simulink model "projectsubaslxcorr"  (R2025a)
settings: Solver=FixedStepAuto  StartTime=0.0  StopTime=0.5  FixedStep=2e-6  RelTol=1e-3
undefined symbols (not defined in the file): dspblkCoreblockFVToolHelper, gcbh
libraries: nesl_utility x21, fl_lib x18, ee_lib x5, simulink x5
settings Model: Creator=Loganathan Mukundhan  LastModifiedBy=msssr

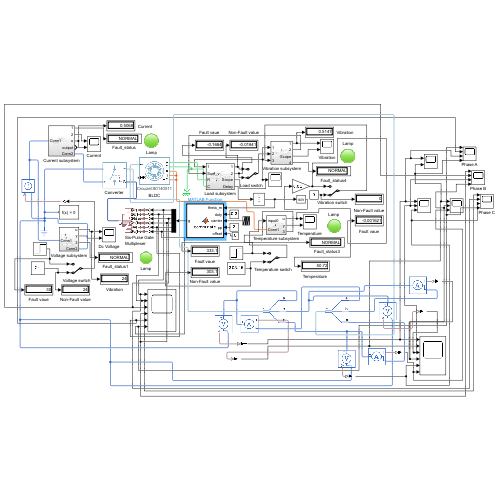
[thumbnail: Simulink's stored preview of the top-level diagram]
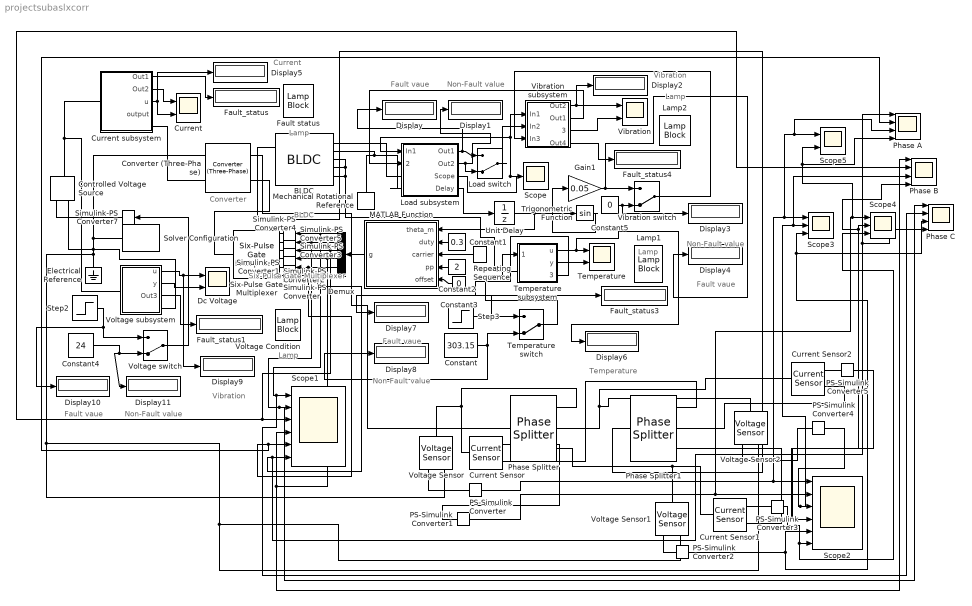
== system projectsubaslxcorr ==
  note: Vibration
  note: Current
  note: Vibration
  note: Fault vaue
  note: Non-Fault value
  note: Temperature
  note: Converter
  note: Six-Pulse Gate
      | Multiplexer
  note: BLDC
  note: Lamp
  note: Lamp
  note: Lamp
  note: Lamp
  note: Non-Fault value
  note: Fault vaue
  note: Non-Fault value
  note: Fault vaue
  note: Non-Fault value
  note: Fault vaue
  BLDC : ee_lib/Electromechanical/Permanent Magnet/BLDC  PartSpecification="{\"CollectionId\":\"SimscapeElectrical\",\"CollectionVersion\":\"1.0.0\",\"DatasetId\":\"Crouzet|80140511|simscape.electrical.bldc\",\"DisplayName\":\"Crouzet:80140511\"}"  port_option=ee.enum.threePhasePort.composite  rotor_param=ee.enum.pmsm.backemf.trapezoidflux  pm_flux_linkage=0.0384885225157163 % Datasheet derived Wb  theta_constant=60 % Assumed angle deg  emf_max=9.6 % Parameter not set V  w_meas=600 % Parameter not set rpm  DphiDtheta_tab=[0, -.1528, -.1528, .1528, .1528, 0] % Parameter not set Wb/rad  back_emf_tab=[0, -9.6, -9.6, 9.6, 9.6, 0] % Parameter not set V  rotor_angle_tab=[0, 7.5, 22.5, 37.5, 52.5, 60] % Parameter not set deg  nPolePairs=2 % Datasheet derived  axes_param=ee.enum.rotorangle.qaxis  winding_type=ee.enum.statorconnection.delta  stator_param=ee.enum.statorparam.LdLqL0  machine_param=ee.enum.dqparameterization.constant  Ld=3.15 % Datasheet derived mH  Lq=3.15 % Datasheet derived mH  idVec=[-200, 0, 200] % Parameter not set A  iqVec=[-200, 0, 200] % Parameter not set A  LdMatrix=0.00022 * ones(3, 3) % Parameter not set H  LqMatrix=0.00022 * ones(3, 3) % Parameter not set H  L0=3.15 % Assumed inductance value mH  Ls=Ls % Parameter not set H  Lm=0 % Parameter not set H  Ms=Ms % Parameter not set H  Rs=1.545 % Datasheet derived Ohm  zero_sequence=ee.enum.park.zerosequence.exclude  loss_param=ee.enum.ironloss.none  losses_oc=[0, 0, 0] % Parameter not set W  losses_sc=[0, 0, 0] % Parameter not set W  f_losses=60 % Parameter not set Hz  Isc_losses=95 % Parameter not set A  J=5e-06 % Datasheet derived kg*m^2  lam=0 % Parameter not set N*m/(rad/s)  i_d_specify=off  i_d_priority=None  i_d=0 A  i_d_nominal_specify=off  i_d_nominal_value=1  i_d_nominal_unit=A  i_q_specify=off  i_q_priority=None  i_q=0 A  i_q_nominal_specify=off  i_q_nominal_value=1  i_q_nominal_unit=A  torque_specify=off  torque_priority=None  torque=0 N*m  torque_nominal_specify=off  torque_nominal_value=1  torque_nominal_unit=N*m  angular_velocity_specify=off  angular_velocity_priority=High  angular_velocity=0 rpm  angular_velocity_nominal_specify=off  angular_velocity_nominal_value=1  angular_velocity_nominal_unit=rpm  angular_position_specify=off  angular_position_priority=High  angular_position=0 deg  angular_position_nominal_specify=off  angular_position_nominal_value=1  angular_position_nominal_unit=deg  alpha=0.00393 % Parameter not set 1/K  alpha_flux=-0.001 % Parameter not set 1/K  Tmeas=298.15 % Parameter not set K  stator_thermal_mass=0.02 J/K  rotor_thermal_mass=0.05 J/K  Rm_percent_rotor=90  Rd_percent_rotor=30  temperatureA_specify=off  temperatureA_priority=High  temperatureA=25 degC  temperatureA_nominal_specify=off  temperatureA_nominal_value=1  temperatureA_nominal_unit=degC  temperatureB_specify=off  temperatureB_priority=High  temperatureB=25 degC  temperatureB_nominal_specify=off  temperatureB_nominal_value=1  temperatureB_nominal_unit=degC  temperatureC_specify=off  temperatureC_priority=High  temperatureC=25 degC  temperatureC_nominal_specify=off  temperatureC_nominal_value=1  temperatureC_nominal_unit=degC  temperatureR_specify=off  temperatureR_priority=High  temperatureR=25 degC  temperatureR_nominal_specify=off  temperatureR_nominal_value=1  temperatureR_nominal_unit=degC
      settings: AttributesFormatString=Crouzet:80140511  InternalSimscapePortConfiguration="{\"Bottom\":[],\"Left\":[{\"id\":\"N\",\"label\":\"~\",\"type\":\"foundation.electrical.three_phase\"},{\"id\":\"HR\",\"label\":\"HR\",\"type\":\"foundation.thermal.thermal\"}],\"Right\":[{\"id\":\"R\",\"label\":\"R\",\"type\":\"foundation.mechanical.rotational.rotational\"},{\"id\":\"C\",\"label\":\"C\",\"type\":\"foundation.mechanical.rotational.rotational\"},{\"id\":\"HA\",\"label\":\"HA\",\"type\":\"foundation.thermal.thermal\"},{\"id\":\"HB\",\"label\":\"HB\",\"type\":\"foundation.thermal.thermal\"},{\"id\":\"HC\",\"label\":\"HC\",\"type\":\"foundation.thermal.thermal\"}],\"Top\":[]}"
  Constant : Constant  Value=303.15
  Constant1 : Constant  Value=0.3
  Constant2 : Constant  Value=2
  Constant3 : Constant  Value=0
  Constant4 : Constant  Value=24
  Constant5 : Constant  Value=0
  Controlled Voltage Source : fl_lib/Electrical/Electrical Sources/Controlled Voltage Source
  Converter (Three-Phase) : ee_lib/Semiconductors & Converters/Converters/Converter (Three-Phase)  port_option=ee.enum.threePhasePort.composite  fidelity_option=ee.enum.converters.fidelity.detailed  device_type=ee.enum.converters.switchingdevice.mosfet  showThermalPort=false  K=0  Vth=0.5 V  Vgt=1 V  Vgt_off=-1 V  Ih=1 A  Vf=0.8 V  Ron=0.001 Ohm  Rds=0.001 Ohm  Goff=1e-6 1/Ohm  Eon_scalar=22.86e-3 J  Eoff_scalar=17.14e-3 J  Eoff_natural_commutation=10e-3 J  Voff=300 V  Iout_scalar=600 A  onCurrentMeasDelay=0 s  useCurrentFromPreviousCycle=false  useVoltageFromPreviousCycle=false  diode_param=ee.enum.converters.protectiondiode.nodynamics  diode_Vf=0.8 V  diode_Ron=0.001 Ohm  diode_Goff=1e-5 1/Ohm  diode_C=50 nF  diode_iRM=-235 A  diode_iF=300 A  diode_idot=-50 A/us  diode_trr_param=ee.enum.converters.diodetrr.trr_factor  diode_trr_factor=3  diode_trr=15 us  diode_Qrr=1500 s*uA  diode_rec_loss_model=ee.enum.diode.reverseRecoveryModel.fixed  diode_ErecVal=0 J  diode_scaleWithIandV=false  diode_ErecMat=zeros(2, 3) J  diode_TjrecVec=[298.15, 398.15] K  diode_IfrecVec=[.1, 1, 10] A  diode_IrecVal=10 A  diode_VrecVal=10 V  diode_tFilter=1 / 1000 / 100 s  thermal_network_parameterization=ee.enum.thermalNetworkTopology.external  Rth=[.08, .5] K/W  Rth_Cauer=[.08, .1, .5] K/W  Rth_Foster=[.08, .14, .22, .16] K/W  thermal_mass_parameterization=ee.enum.thermalNetwork.timeconstant  thermal_mass=[.01, .5] J/K  thermal_mass_Cauer=[.01, .1, .5] J/K  thermal_mass_Foster=[.001, .005, .05, .5] J/K  thermal_time_constant=[.001, .2] s  thermal_time_constant_Cauer=[.001, .1, .2] s  thermal_time_constant_Foster=[7e-05, .0007, .01, .08] s  thermal_mass_initial_temperatures=[25, 25] degC  thermal_mass_initial_temperatures_Cauer=[25, 25, 25] degC  junction_thermal_mass=0.01 J/K  Tvec_initial_Foster=[25, 25, 25, 25] degC  snubber_type=ee.enum.converters.snubber.exclude  Cs=1e-7 F  Rs=0.1 Ohm  Vce_loss=[0, 150, 300] V
  Current : Scope  NumInputPorts=2
      settings: ActiveDisplayYMinimum=-0.12499999999999997  ActiveDisplayYMaximum=1.125  DataLoggingVariableName=ScopeData3
  Current Sensor : fl_lib/Electrical/Electrical Sensors/Current Sensor
  Current Sensor1 : fl_lib/Electrical/Electrical Sensors/Current Sensor
  Current Sensor2 : fl_lib/Electrical/Electrical Sensors/Current Sensor
  Current subsystem : Subsystem
  Dc Voltage : Scope  NumInputPorts=2
      settings: ActiveDisplayYMinimum=-1  ActiveDisplayYMaximum=1  DataLoggingVariableName=ScopeData4
  Demux : Demux  Outputs=6
  Display{,1..11} (12 alike) : Display
  Electrical Reference : fl_lib/Electrical/Electrical Elements/Electrical Reference
  Fault status : LampBlock  LabelPosition=Hide  DefaultColor=[192.0, 192.0, 192.0]
  Fault_status{,1,3..4} (4 alike) : Display
  Gain1 : Gain  Gain=0.05
  Lamp1 : LampBlock  LabelPosition=Hide  DefaultColor=[192.0, 192.0, 192.0]
  Lamp2 : LampBlock  LabelPosition=Hide  DefaultColor=[192.0, 192.0, 192.0]
  Load subsystem : Subsystem
  Load switch : ManualSwitch  CurrentSetting=0
  MATLAB Function : MATLAB Function  TreatAsAtomicUnit=on
  Mechanical Rotational Reference : fl_lib/Mechanical/Rotational Elements/Mechanical Rotational Reference
  PS-Simulink Converter{,1..5} (6 alike) : nesl_utility/PS-Simulink Converter  PhysicalDomain=network_engine_domain  SubClassName=ps_output  LeftPortType=input  RightPortType=output  PseudoPeriodic=off  Frequencies=[]  VectorFormat=inherit  Unit=inherit  AffineConversion=off
  Phase A : Scope  NumInputPorts=4
      settings: ActiveDisplayYMinimum=-0.012079831932773066  ActiveDisplayYMaximum=1.0252100840336134  DataLoggingVariableName=ScopeData10
  Phase B : Scope  NumInputPorts=4
      settings: ActiveDisplayYMinimum=-0.12499999999999997  ActiveDisplayYMaximum=1.125  DataLoggingVariableName=ScopeData11
  Phase C : Scope  NumInputPorts=4
      settings: ActiveDisplayYMinimum=-0.031775210084033612  ActiveDisplayYMaximum=1.0317752100840336  DataLoggingVariableName=ScopeData12
  Phase Splitter : ee_lib/Connectors & References/Phase Splitter
  Phase Splitter1 : ee_lib/Connectors & References/Phase Splitter
  Repeating Sequence : simulink/Sources/Repeating Sequence  rep_seq_t=[0 1e-4]  rep_seq_y=[0 1]
  Scope : Scope
      settings: ActiveDisplayYMinimum=-12.045945676542038  ActiveDisplayYMaximum=108.41351108887838
  Scope1 : Scope  NumInputPorts=6
      settings: ActiveDisplayYMinimum=-0.12499999999999997  ActiveDisplayYMaximum=1.125
  Scope2 : Scope  NumInputPorts=6
      settings: ActiveDisplayYMinimum=-1.7770072942224644  ActiveDisplayYMaximum=27.088124454668268  DataLoggingVariableName=ScopeData2
  Scope3 : Scope  NumInputPorts=3
      settings: ActiveDisplayYMinimum=-2.8282937021531112  ActiveDisplayYMaximum=26.5262867042067  DataLoggingVariableName=ScopeData5
  Scope4 : Scope  NumInputPorts=3
      settings: DataLoggingVariableName=ScopeData7
  Scope5 : Scope  NumInputPorts=2
      settings: ActiveDisplayYMinimum=-1.0622016680044801  ActiveDisplayYMaximum=26.229780400571709  DataLoggingVariableName=ScopeData9
  Simulink-PS Converter{,1..5,7} (7 alike) : nesl_utility/Simulink-PS Converter  PhysicalDomain=network_engine_domain  SubClassName=ps_input  LeftPortType=input  RightPortType=output  PseudoPeriodic=off  Frequencies=[]  NoiseDistribution=none  NoiseParameters=[]  Unit=1  AffineConversion=off  FilteringAndDerivatives=provide  SimscapeFilterOrder=1  InputFilterTimeConstant=0.001  UdotUserProvided=0
  Six-Pulse Gate Multiplexer : ee_lib/Semiconductors & Converters/Converters/Six-Pulse Gate Multiplexer  port_option=ee.enum.controlport.ps
  Solver Configuration : nesl_utility/Solver Configuration  PhysicalDomain=network_engine_domain  SubClassName=solver  LeftPortType=input  RightPortType=generic  Tones=[]  Harmonics=[]  SimulateNoise=off  Profile=off  UseLocalSampling=off  EnableSwitchedLinearOptims=on  FrequencyDomain=off  UseCCode=off  RelTol=0.001  AbsTol=0.001  MinStep=1e-09  ToWorkspace=off  RevertToSquareIcSolve=off  NumHomotopyIterations=100  PhasorMode=off  PhasorModeNumHarmonics=1  ConsistencySolver=NEWTON_XTOL_AFTER_FTOL  IndexReductionMethod=DerivativeReplacement  DoDC=off  ResidualTolerance=1e-09  ConsistencyTolSource=GLOBAL  ConsistencyAbsTol=0.001  ConsistencyRelTol=0.001  ConsistencyTolFactor=0.001  UseLocalSolver=on  LocalSolverChoice=NE_BACKWARD_EULER_ADVANCER  ResolveIndetEquations=on  FunctionEvalNumThread=1  LocalSolverSampleTime=2e-6  DoFixedCost=off  MaxNonlinIter=3  MaxModeIter=2  ComputeImpulses=off  ImpulseIterations=2  LinearAlgebra=auto  LinearAlgebraNumThread=0  EquationFormulation=NE_TIME_EF  DelaysMemoryBudget=1024  AutomaticFiltering=on  FilteringTimeConstant=0.001  PartitionStorageMethod=AS_NEEDED  PartitionMemoryBudget=1024  PartitionMethod=ROBUST  MultibodyUseLocalSolver=off  MultibodyLocalSolverChoice=ODE1  MultibodyLocalSolverSampleTime=0.001
  Step2 : Step  Time=0.25  Before=24  After=30  SampleTime=0
  Step3 : Step  Time=0.25  Before=303.15  After=333.15  SampleTime=0
  Temperature : Scope  NumInputPorts=2
      settings: ActiveDisplayYMinimum=13.049582437412266  ActiveDisplayYMaximum=132.55375806328965  DataLoggingVariableName=ScopeData6
  Temperature subsystem : Subsystem
  Temperature switch : ManualSwitch  CurrentSetting=0
  Trigonometric Function : Trigonometry
  Unit Delay : UnitDelay  SampleTime=2e-6  HasFrameUpgradeWarning=on
  Vibration : Scope  NumInputPorts=2
      settings: ActiveDisplayYMinimum=-2.0330445480545611  ActiveDisplayYMaximum=18.297400932491055  DataLoggingVariableName=ScopeData8
  Vibration subsystem : Subsystem
  "Vibration switch  " : ManualSwitch  CurrentSetting=0
  Voltage Condition : LampBlock  LabelPosition=Hide  DefaultColor=[192.0, 192.0, 192.0]
  Voltage Sensor : fl_lib/Electrical/Electrical Sensors/Voltage Sensor
  Voltage Sensor1 : fl_lib/Electrical/Electrical Sensors/Voltage Sensor
  Voltage Sensor2 : fl_lib/Electrical/Electrical Sensors/Voltage Sensor
  Voltage subsystem : Subsystem
  Voltage switch : ManualSwitch  CurrentSetting=0
  wires:
  Demux/1 -> Phase C/2, Scope1/1, Simulink-PS Converter5/1
  Demux/2 -> Phase C/1, Scope1/2, Simulink-PS Converter4/1
  Demux/3 -> Scope1/3, Phase B/2, Simulink-PS Converter3/1
  Demux/4 -> Scope1/4, Phase B/1, Simulink-PS Converter2/1
  Demux/5 -> Phase A/2, Scope1/5, Simulink-PS Converter1/1
  Demux/6 -> Phase C/4, Phase A/1, Scope1/6, Simulink-PS Converter/1
  MATLAB Function/1(g) -> Demux/1
  Constant3/1 -> MATLAB Function/5(offset)
  Constant1/1 -> MATLAB Function/2(duty)
  Constant2/1 -> MATLAB Function/4(pp)
  Repeating Sequence/1 -> MATLAB Function/3(carrier)
  Step2/1 -> Display10/1, Voltage switch/1
  Constant4/1 -> Voltage switch/2, Display11/1
  Step3/1 -> Display7/1, Temperature switch/1
  Constant/1 -> Temperature switch/2, Display8/1
  Constant5/1 -> Display3/1, "Vibration switch  "/2
  Unit Delay/1 -> Trigonometric Function/1, MATLAB Function/1(theta_m)
  Trigonometric Function/1 -> Gain1/1
  Gain1/1 -> Display4/1, "Vibration switch  "/1
  Current subsystem/1(Out1) -> Fault_status/1
  Current subsystem/2(Out2) -> Current/1
  Current subsystem/3(u) -> Current/2, Display5/1
  Voltage subsystem/1(u) -> Display9/1, Dc Voltage/1
  Voltage subsystem/3(Out3) -> Fault_status1/1
  Load subsystem/3(Scope) -> Vibration subsystem/1(In1), Load subsystem/1(In1), Scope/1
  Load subsystem/1(Out1) -> Display/1, Load switch/1
  Load subsystem/2(Out2) -> Display1/1, Load switch/2
  Load subsystem/4(Delay) -> Unit Delay/1
  Temperature switch/1 -> Temperature subsystem/1(input0)
  Temperature subsystem/1(u) -> Display6/1, Temperature/1
  Temperature subsystem/2(y) -> Temperature/2
  Temperature subsystem/3(Out3) -> Fault_status3/1
  Load switch/1 -> Vibration subsystem/2(In2)
  "Vibration switch  "/1 -> Vibration subsystem/3(In3)
  Vibration subsystem/2(Out1) -> Load subsystem/2(Sum_v)
  Vibration subsystem/1(Out2) -> Vibration/1, Display2/1
  Vibration subsystem/3(Scope) -> Vibration/2
  Vibration subsystem/4(Out4) -> Fault_status4/1
  Voltage switch/1 -> Simulink-PS Converter7/1
  Voltage subsystem/2(y) -> Dc Voltage/2
  PS-Simulink Converter/1 -> Phase A/3, Scope5/1, Scope3/1, Scope2/1
  PS-Simulink Converter1/1 -> Scope2/2, Phase A/4, Scope5/2, Scope4/1
  PS-Simulink Converter4/1 -> Phase B/3, Scope3/2, Scope2/3
  PS-Simulink Converter5/1 -> Scope2/4, Scope4/2, Phase B/4
  PS-Simulink Converter2/1 -> Scope2/5, Phase C/3, Scope3/3
  PS-Simulink Converter3/1 -> Scope4/3, Scope2/6
  connections:
  Solver Configuration/RConn1 -- Voltage Sensor1/RConn2 -- Voltage Sensor2/RConn2 -- Voltage Sensor/RConn2 -- Electrical Reference/LConn1 -- Controlled Voltage Source/RConn2 -- Voltage subsystem/RConn1 -- Converter (Three-Phase)/RConn2
  Six-Pulse Gate Multiplexer/RConn1 -- Converter (Three-Phase)/LConn1
  Simulink-PS Converter5/RConn1 -- Six-Pulse Gate Multiplexer/LConn6
  Simulink-PS Converter4/RConn1 -- Six-Pulse Gate Multiplexer/LConn5
  Simulink-PS Converter3/RConn1 -- Six-Pulse Gate Multiplexer/LConn4
  Simulink-PS Converter2/RConn1 -- Six-Pulse Gate Multiplexer/LConn3
  Simulink-PS Converter1/RConn1 -- Six-Pulse Gate Multiplexer/LConn2
  Simulink-PS Converter/RConn1 -- Six-Pulse Gate Multiplexer/LConn1
  Mechanical Rotational Reference/LConn1 -- Load subsystem/LConn2 -- BLDC/RConn2
  Controlled Voltage Source/LConn1 -- Current subsystem/LConn1 -- Voltage subsystem/LConn1
  Simulink-PS Converter7/RConn1 -- Controlled Voltage Source/RConn1
  BLDC/RConn3 -- Temperature subsystem/LConn1 -- BLDC/RConn5 -- BLDC/RConn4
  Current subsystem/RConn1 -- Converter (Three-Phase)/RConn1
  Load subsystem/LConn1 -- BLDC/RConn1
  Converter (Three-Phase)/LConn2 -- Phase Splitter/LConn1
  Phase Splitter1/LConn1 -- BLDC/LConn1
  Voltage Sensor/RConn1 -- PS-Simulink Converter/LConn1
  Current Sensor/RConn1 -- PS-Simulink Converter1/LConn1
  Phase Splitter/RConn1 -- Voltage Sensor/LConn1 -- Current Sensor/LConn1
  Current Sensor/RConn2 -- Phase Splitter1/RConn1
  Phase Splitter/RConn2 -- Voltage Sensor2/LConn1 -- Current Sensor2/LConn1
  Current Sensor2/RConn2 -- Phase Splitter1/RConn2
  Phase Splitter/RConn3 -- Voltage Sensor1/LConn1 -- Current Sensor1/LConn1
  Current Sensor1/RConn2 -- Phase Splitter1/RConn3
  PS-Simulink Converter2/LConn1 -- Voltage Sensor1/RConn1
  PS-Simulink Converter3/LConn1 -- Current Sensor1/RConn1
  PS-Simulink Converter4/LConn1 -- Voltage Sensor2/RConn1
  PS-Simulink Converter5/LConn1 -- Current Sensor2/RConn1

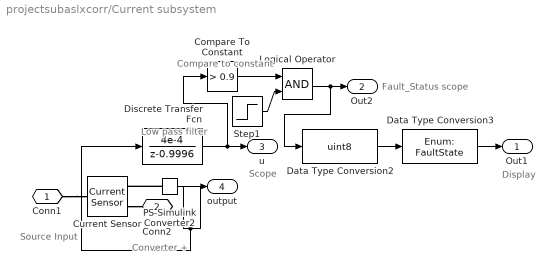
== system projectsubaslxcorr/Current subsystem ==
  note: Display
  note: Scope
  note: Fault_Status scope
  note: Converter +
  note: Source Input
  note: Compare to constant
  note: Low pass filter
  Compare To Constant : simulink/Logic and Bit Operations/Compare To Constant  relop=>  const=0.9  OutDataTypeStr=boolean
  Current Sensor : fl_lib/Electrical/Electrical Sensors/Current Sensor
  Data Type Conversion2 : DataTypeConversion  OutDataTypeStr=uint8  SaturateOnIntegerOverflow=off  RndMeth=Floor
  Data Type Conversion3 : DataTypeConversion  OutDataTypeStr=Enum: FaultState  SaturateOnIntegerOverflow=off  RndMeth=Floor
  Discrete Transfer Fcn : DiscreteTransferFcn  LoadFcn=dspblkCoreblockFVToolHelper(gcbh,'load');  Numerator=[4e-4]  Denominator=[1 -0.9996]
      settings: CopyFcn=dspblkCoreblockFVToolHelper(gcbh,'copy');  DeleteFcn=dspblkCoreblockFVToolHelper(gcbh,'close');  ModelCloseFcn=dspblkCoreblockFVToolHelper(gcbh,'close');  PreSaveFcn=dspblkCoreblockFVToolHelper(gcbh,'presave');  PostSaveFcn=dspblkCoreblockFVToolHelper(gcbh,'postsave');  CloseFcn=dspblkCoreblockFVToolHelper(gcbh,'close');
  Logical Operator : Logic  AllPortsSameDT=off  OutDataTypeStr=boolean
  PS-Simulink Converter2 : nesl_utility/PS-Simulink Converter  PhysicalDomain=network_engine_domain  SubClassName=ps_output  LeftPortType=input  RightPortType=output  PseudoPeriodic=off  Frequencies=[]  VectorFormat=inherit  Unit=inherit  AffineConversion=off
  Step1 : Step  Time=0.1  SampleTime=0
  Conn1 : PMIOPort  Side=Left
  Conn2 : PMIOPort  Port=2  Side=Right
  Out1 : Outport
  Out2 : Outport  Port=2
  u : Outport  Port=3
  output : Outport  Port=4
  wires:
  PS-Simulink Converter2/1 -> output/1, Discrete Transfer Fcn/1
  Logical Operator/1 -> Out2/1, Data Type Conversion2/1
  Compare To Constant/1 -> Logical Operator/1
  Discrete Transfer Fcn/1 -> Compare To Constant/1, u/1
  Data Type Conversion3/1 -> Out1/1
  Data Type Conversion2/1 -> Data Type Conversion3/1
  Step1/1 -> Logical Operator/2
  connections:
  PS-Simulink Converter2/LConn1 -- Current Sensor/RConn1
  Current Sensor/RConn2 -- Conn2/RConn1
  Conn1/RConn1 -- Current Sensor/LConn1

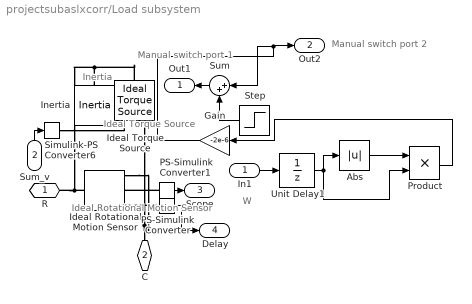
== system projectsubaslxcorr/Load subsystem ==
  note: W
  note: Manual switch port 2
  note: Ideal Rotational
      | Motion Sensor
  note: Ideal Torque
      | Source
  note: Inertia
  note: Manual switch port 1
  In1 : Inport
  Sum_v : Inport  Port=2
  Abs : Abs  SaturateOnIntegerOverflow=off
  Gain : Gain  Gain=-2e-6
  Ideal Rotational Motion Sensor : fl_lib/Mechanical/Mechanical Sensors/Ideal Rotational Motion Sensor  reference=foundation.enum.MeasurementReference.difference  acceleration_port=false  velocity_port=true  position_port=true  wrap_angle=false  offset=0 rad
  Ideal Torque Source : fl_lib/Mechanical/Mechanical Sources/Ideal Torque Source
  Inertia : fl_lib/Mechanical/Rotational Elements/Inertia  inertia=1e-4 kg*m^2  num_ports=foundation.enum.numPorts2.one  w_specify=off  w_priority=High  w=0 rad/s  w_nominal_specify=off  w_nominal_value=1  w_nominal_unit=rad/s  t_specify=off  t_priority=None  t=0 N*m  t_nominal_specify=off  t_nominal_value=1  t_nominal_unit=N*m
  PS-Simulink Converter : nesl_utility/PS-Simulink Converter  PhysicalDomain=network_engine_domain  SubClassName=ps_output  LeftPortType=input  RightPortType=output  PseudoPeriodic=off  Frequencies=[]  VectorFormat=inherit  Unit=inherit  AffineConversion=off
  PS-Simulink Converter1 : nesl_utility/PS-Simulink Converter  PhysicalDomain=network_engine_domain  SubClassName=ps_output  LeftPortType=input  RightPortType=output  PseudoPeriodic=off  Frequencies=[]  VectorFormat=inherit  Unit=inherit  AffineConversion=off
  Product : Product
  Simulink-PS Converter6 : nesl_utility/Simulink-PS Converter  PhysicalDomain=network_engine_domain  SubClassName=ps_input  LeftPortType=input  RightPortType=output  PseudoPeriodic=off  Frequencies=[]  NoiseDistribution=none  NoiseParameters=[]  Unit=1  AffineConversion=off  FilteringAndDerivatives=provide  SimscapeFilterOrder=1  InputFilterTimeConstant=0.001  UdotUserProvided=0
  Step : Step  Time=0.25  After=-0.15  SampleTime=0
  Sum : Sum  Inputs=|++
  Unit Delay1 : UnitDelay  SampleTime=2e-6  HasFrameUpgradeWarning=on
  R : PMIOPort  Side=Left
  C : PMIOPort  Port=2  Side=Left
  Out1 : Outport
  Out2 : Outport  Port=2
  Scope : Outport  Port=3
  Delay : Outport  Port=4
  wires:
  Unit Delay1/1 -> Abs/1, Product/2
  Abs/1 -> Product/1
  Product/1 -> Gain/1
  Step/1 -> Sum/2
  Gain/1 -> Out2/1, Sum/1
  Sum/1 -> Out1/1
  PS-Simulink Converter/1 -> Delay/1
  Sum_v/1 -> Simulink-PS Converter6/1
  In1/1 -> Unit Delay1/1
  PS-Simulink Converter1/1 -> Scope/1
  connections:
  Ideal Rotational Motion Sensor/RConn1 -- Ideal Torque Source/RConn2 -- C/RConn1
  PS-Simulink Converter/LConn1 -- Ideal Rotational Motion Sensor/RConn3
  Ideal Rotational Motion Sensor/LConn1 -- Ideal Torque Source/LConn1 -- Inertia/LConn1 -- R/RConn1
  Simulink-PS Converter6/RConn1 -- Ideal Torque Source/RConn1
  PS-Simulink Converter1/LConn1 -- Ideal Rotational Motion Sensor/RConn2

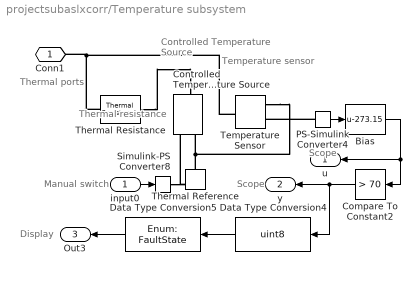
== system projectsubaslxcorr/Temperature subsystem ==
  note: Scope
  note: Display
  note: Thermal ports
  note: Manual switch
  note: Temperature
      | sensor
  note: Controlled
      | Temperature
      | Source
  note: Thermal resistance
  note: Scope
  input0 : Inport
  Bias : Bias  Bias=-273.15  SaturateOnIntegerOverflow=off
  Compare To Constant2 : simulink/Logic and Bit Operations/Compare To Constant  relop=>  const=70  OutDataTypeStr=boolean
  Controlled Temperature Source : fl_lib/Thermal/Thermal Sources/Controlled Temperature Source
  Data Type Conversion4 : DataTypeConversion  OutDataTypeStr=uint8  SaturateOnIntegerOverflow=off  RndMeth=Floor
  Data Type Conversion5 : DataTypeConversion  OutDataTypeStr=Enum: FaultState  SaturateOnIntegerOverflow=off  RndMeth=Floor
  PS-Simulink Converter4 : nesl_utility/PS-Simulink Converter  PhysicalDomain=network_engine_domain  SubClassName=ps_output  LeftPortType=input  RightPortType=output  PseudoPeriodic=off  Frequencies=[]  VectorFormat=inherit  Unit=inherit  AffineConversion=off
  Simulink-PS Converter8 : nesl_utility/Simulink-PS Converter  PhysicalDomain=network_engine_domain  SubClassName=ps_input  LeftPortType=input  RightPortType=output  PseudoPeriodic=off  Frequencies=[]  NoiseDistribution=none  NoiseParameters=[]  Unit=1  AffineConversion=off  FilteringAndDerivatives=provide  SimscapeFilterOrder=1  InputFilterTimeConstant=0.001  UdotUserProvided=0
  Temperature Sensor : fl_lib/Thermal/Thermal Sensors/Temperature Sensor  temperature_measure=foundation.enum.MeasurementReference.difference
  Thermal Reference : fl_lib/Thermal/Thermal Elements/Thermal Reference
  Thermal Resistance : fl_lib/Thermal/Thermal Elements/Thermal Resistance  resistance=2 K/W  T_specify=off  T_priority=None  T=0 K  T_nominal_specify=off  T_nominal_value=1  T_nominal_unit=K  Q_specify=off  Q_priority=None  Q=0 W  Q_nominal_specify=off  Q_nominal_value=1  Q_nominal_unit=W
  Conn1 : PMIOPort  Side=Left
  u : Outport
  y : Outport  Port=2
  Out3 : Outport  Port=3
  wires:
  Data Type Conversion4/1 -> Data Type Conversion5/1
  PS-Simulink Converter4/1 -> Bias/1
  Compare To Constant2/1 -> Data Type Conversion4/1, y/1
  input0/1 -> Simulink-PS Converter8/1
  Bias/1 -> Compare To Constant2/1, u/1
  Data Type Conversion5/1 -> Out3/1
  connections:
  Temperature Sensor/LConn1 -- Conn1/RConn1 -- Thermal Resistance/LConn1
  Thermal Reference/LConn1 -- Temperature Sensor/RConn1 -- Controlled Temperature Source/RConn2
  Thermal Resistance/RConn1 -- Controlled Temperature Source/LConn1
  PS-Simulink Converter4/LConn1 -- Temperature Sensor/RConn2
  Simulink-PS Converter8/RConn1 -- Controlled Temperature Source/RConn1

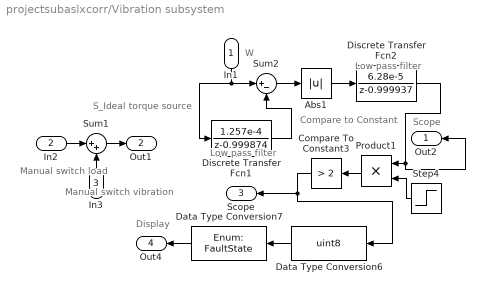
== system projectsubaslxcorr/Vibration subsystem ==
  note: W
  note: Manual switch
      | load
  note: Scope
  note: Display
  note: S_Ideal torque source
  note: Compare to
      | Constant
  note: Low pass filter
  note: Low pass filter
  note: Manual switch
      | vibration
  In1 : Inport
  In2 : Inport  Port=2
  In3 : Inport  Port=3
  Abs1 : Abs  SaturateOnIntegerOverflow=off
  Compare To Constant3 : simulink/Logic and Bit Operations/Compare To Constant  relop=>  const=2  OutDataTypeStr=boolean
  Data Type Conversion6 : DataTypeConversion  OutDataTypeStr=uint8  SaturateOnIntegerOverflow=off  RndMeth=Floor
  Data Type Conversion7 : DataTypeConversion  OutDataTypeStr=Enum: FaultState  SaturateOnIntegerOverflow=off  RndMeth=Floor
  Discrete Transfer Fcn1 : DiscreteTransferFcn  LoadFcn=dspblkCoreblockFVToolHelper(gcbh,'load');  Numerator=[1.257e-4]  Denominator=[1 -0.999874]
      settings: CopyFcn=dspblkCoreblockFVToolHelper(gcbh,'copy');  DeleteFcn=dspblkCoreblockFVToolHelper(gcbh,'close');  ModelCloseFcn=dspblkCoreblockFVToolHelper(gcbh,'close');  PreSaveFcn=dspblkCoreblockFVToolHelper(gcbh,'presave');  PostSaveFcn=dspblkCoreblockFVToolHelper(gcbh,'postsave');  CloseFcn=dspblkCoreblockFVToolHelper(gcbh,'close');
  Discrete Transfer Fcn2 : DiscreteTransferFcn  LoadFcn=dspblkCoreblockFVToolHelper(gcbh,'load');  Numerator=[6.28e-5]  Denominator=[1 -0.999937]
      settings: CopyFcn=dspblkCoreblockFVToolHelper(gcbh,'copy');  DeleteFcn=dspblkCoreblockFVToolHelper(gcbh,'close');  ModelCloseFcn=dspblkCoreblockFVToolHelper(gcbh,'close');  PreSaveFcn=dspblkCoreblockFVToolHelper(gcbh,'presave');  PostSaveFcn=dspblkCoreblockFVToolHelper(gcbh,'postsave');  CloseFcn=dspblkCoreblockFVToolHelper(gcbh,'close');
  Product1 : Product
  Step4 : Step  Time=0.25  SampleTime=0
  Sum1 : Sum  Inputs=|++
  Sum2 : Sum  Inputs=|+-
  Out2 : Outport
  Out1 : Outport  Port=2
  Scope : Outport  Port=3
  Out4 : Outport  Port=4
  wires:
  Data Type Conversion6/1 -> Data Type Conversion7/1
  Discrete Transfer Fcn2/1 -> Out2/1, Product1/1
  Abs1/1 -> Discrete Transfer Fcn2/1
  Sum1/1 -> Out1/1
  Product1/1 -> Compare To Constant3/1
  Discrete Transfer Fcn1/1 -> Sum2/2
  Step4/1 -> Product1/2
  Compare To Constant3/1 -> Scope/1, Data Type Conversion6/1
  In1/1 -> Sum2/1, Discrete Transfer Fcn1/1
  Sum2/1 -> Abs1/1
  In2/1 -> Sum1/1
  In3/1 -> Sum1/2
  Data Type Conversion7/1 -> Out4/1

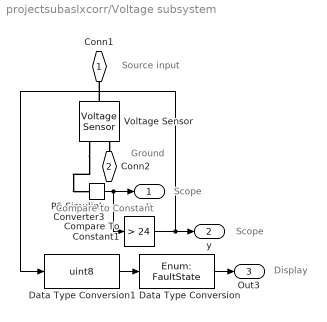
== system projectsubaslxcorr/Voltage subsystem ==
  note: Display
  note: Scope
  note: Ground
  note: Source input
  note: Compare to
      | Constant
  note: Scope
  Compare To Constant1 : simulink/Logic and Bit Operations/Compare To Constant  relop=>  const=24  OutDataTypeStr=boolean
  Data Type Conversion : DataTypeConversion  OutDataTypeStr=Enum: FaultState  SaturateOnIntegerOverflow=off  RndMeth=Floor
  Data Type Conversion1 : DataTypeConversion  OutDataTypeStr=uint8  SaturateOnIntegerOverflow=off  RndMeth=Floor
  PS-Simulink Converter3 : nesl_utility/PS-Simulink Converter  PhysicalDomain=network_engine_domain  SubClassName=ps_output  LeftPortType=input  RightPortType=output  PseudoPeriodic=off  Frequencies=[]  VectorFormat=inherit  Unit=inherit  AffineConversion=off
  Voltage Sensor : fl_lib/Electrical/Electrical Sensors/Voltage Sensor
  Conn1 : PMIOPort  Side=Left
  Conn2 : PMIOPort  Port=2  Side=Right
  u : Outport
  y : Outport  Port=2
  Out3 : Outport  Port=3
  wires:
  Compare To Constant1/1 -> y/1, Data Type Conversion1/1
  PS-Simulink Converter3/1 -> u/1, Compare To Constant1/1
  Data Type Conversion1/1 -> Data Type Conversion/1
  Data Type Conversion/1 -> Out3/1
  connections:
  Voltage Sensor/RConn2 -- Conn2/RConn1
  Voltage Sensor/LConn1 -- Conn1/RConn1
  Voltage Sensor/RConn1 -- PS-Simulink Converter3/LConn1

== matlab function projectsubaslxcorr/MATLAB Function ==
  data: theta_m input; g output; duty input; carrier input; pp input; offset input
function g = commutate(theta_m, duty, carrier, pp, offset)
% output order matches your Demux: [CL CH BL BH AL AH]
the = pp*theta_m + offset;
s = floor(mod(the - pi/6, 2*pi)/(pi/3));
s = min(max(s,0),5);
P = [1 1 2 2 3 3];     % phase on high side
N = [2 3 3 1 1 2];     % phase on low side
g = zeros(6,1);        % internal order [AH AL BH BL CH CL]
g(2*P(s+1)-1) = double(duty > carrier);
g(2*N(s+1))   = 1;
g = flipud(g);f
end
